simulink model "Slider_Crank_04_auto"  (R2026b)
settings: Solver=ode15s  StopTime=2  MaxStep=0.001  RelTol=1e-5
model workspace (MAT data in the model file):
  Crank_Radius = 0.015
  Crank_Speed = 12.5663706144
  Dead_Volume = 1e-05
  Initial_Tank_Volume = 0.001
  Piston_Area = 0.001
  Piston_Stroke = 0.05
  Pump_Frequency = 2
  Rod_Length = 0.075
  Tank_Area = 0.02
  Valve_Crack_Pressure = 1000
  Valve_Full_Pressure = 10000
undefined symbols (not defined in the file): X, Y, Z
libraries: sm_lib x15, fl_lib x6, nesl_utility x4, SimscapeFluids_lib x3, simulink x1
settings Model: Creator=smiller  LastModifiedBy=smiller
settings SimscapeCC: SimscapeLogType=all  SimscapeNominalValues="[{\"value\":\"1\",\"unit\":\"A\"},{\"value\":\"1\",\"unit\":\"bar\"},{\"value\":\"1\",\"unit\":\"cm^2\"},{\"value\":\"1\",\"unit\":\"cm^3/s\"},{\"value\":\"1\",\"unit\":\"kJ/kg\"},{\"value\":\"1\",\"unit\":\"kW\"},{\"value\":\"1\",\"unit\":\"l\"},{\"value\":\"1\",\"unit\":\"N\"},{\"value\":\"1\",\"unit\":\"N*m\"},{\"value\":\"1\",\"unit\":\"V\"},{\"value\":\"0.001\",\"unit\":\"Wb\"}]"  SimscapeUseEnergyAccounting=off

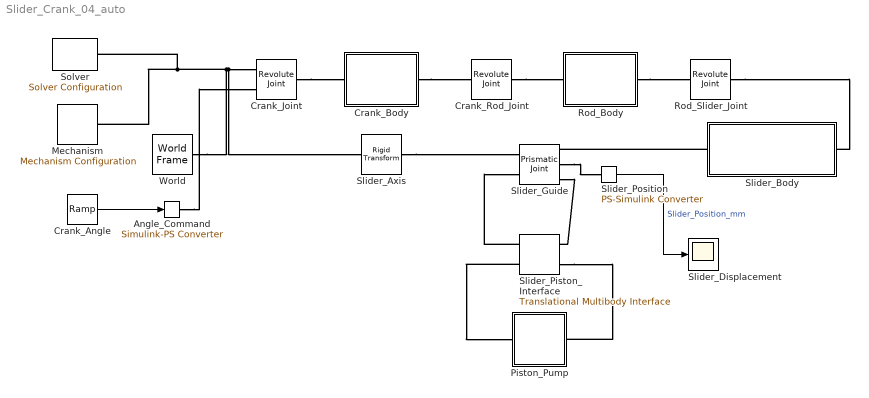
== system Slider_Crank_04_auto ==
  Angle_Command : nesl_utility/Simulink-PS Converter  PhysicalDomain=network_engine_domain  SubClassName=ps_input  LeftPortType=input  RightPortType=output  PseudoPeriodic=off  Frequencies=[]  NoiseDistribution=none  NoiseParameters=[]  Unit=rad  AffineConversion=off  FilteringAndDerivatives=filter  SimscapeFilterOrder=2  InputFilterTimeConstant=0.001  UdotUserProvided=0
  Crank_Angle : simulink/Sources/Ramp  slope=Crank_Speed  start=0  InitialOutput=0
  Crank_Body : Subsystem
  Crank_Joint : sm_lib/Joints/Revolute Joint  JointMode=Normal  CompositeWrenchDir=FollowerOnBase  CompositeWrenchFrame=BaseFrame  SenseConstraintForce=off  SenseConstraintTorque=off  SenseTotalForce=off  SenseTotalTorque=off  PositionTargetSpecify=off  PositionTargetPriority=High  PositionTargetValue=0  PositionTargetValueUnits=deg  VelocityTargetSpecify=off  VelocityTargetPriority=High  VelocityTargetValue=0  VelocityTargetValueUnits=deg/s  EquilibriumPosition=0  EquilibriumPositionUnits=deg  SpringStiffness=0  SpringStiffnessUnits=N*m/deg  DampingCoefficient=0  DampingCoefficientUnits=N*m/(deg/s)  LowerLimitSpecify=off  LowerLimitBound=-90  LowerLimitBoundUnits=deg  LowerLimitStiffness=1e4  LowerLimitStiffnessUnits=N*m/deg  LowerLimitDamping=10  LowerLimitDampingUnits=N*m/(deg/s)  LowerLimitTransitionRegionWidth=0.1  LowerLimitTransitionRegionWidthUnits=deg  UpperLimitSpecify=off  UpperLimitBound=90  UpperLimitBoundUnits=deg  UpperLimitStiffness=1e4  UpperLimitStiffnessUnits=N*m/deg  UpperLimitDamping=10  UpperLimitDampingUnits=N*m/(deg/s)  UpperLimitTransitionRegionWidth=0.1  UpperLimitTransitionRegionWidthUnits=deg  TorqueActuationMode=ComputedTorque  MotionActuationMode=InputMotion  SensePosition=off  SenseVelocity=off  SenseAcceleration=off  SenseTorqueForce=off  SenseLowerLimitTorqueForce=off  SenseUpperLimitTorqueForce=off
  Crank_Rod_Joint : sm_lib/Joints/Revolute Joint  JointMode=Normal  CompositeWrenchDir=FollowerOnBase  CompositeWrenchFrame=BaseFrame  SenseConstraintForce=off  SenseConstraintTorque=off  SenseTotalForce=off  SenseTotalTorque=off  PositionTargetSpecify=off  PositionTargetPriority=High  PositionTargetValue=0  PositionTargetValueUnits=deg  VelocityTargetSpecify=off  VelocityTargetPriority=High  VelocityTargetValue=0  VelocityTargetValueUnits=deg/s  EquilibriumPosition=0  EquilibriumPositionUnits=deg  SpringStiffness=0  SpringStiffnessUnits=N*m/deg  DampingCoefficient=0  DampingCoefficientUnits=N*m/(deg/s)  LowerLimitSpecify=off  LowerLimitBound=-90  LowerLimitBoundUnits=deg  LowerLimitStiffness=1e4  LowerLimitStiffnessUnits=N*m/deg  LowerLimitDamping=10  LowerLimitDampingUnits=N*m/(deg/s)  LowerLimitTransitionRegionWidth=0.1  LowerLimitTransitionRegionWidthUnits=deg  UpperLimitSpecify=off  UpperLimitBound=90  UpperLimitBoundUnits=deg  UpperLimitStiffness=1e4  UpperLimitStiffnessUnits=N*m/deg  UpperLimitDamping=10  UpperLimitDampingUnits=N*m/(deg/s)  UpperLimitTransitionRegionWidth=0.1  UpperLimitTransitionRegionWidthUnits=deg  TorqueActuationMode=NoTorque  MotionActuationMode=ComputedMotion  SensePosition=off  SenseVelocity=off  SenseAcceleration=off  SenseTorqueForce=off  SenseLowerLimitTorqueForce=off  SenseUpperLimitTorqueForce=off
  Mechanism : sm_lib/Utilities/Mechanism Configuration  UniformGravity=Constant  GravityVector=[0 -9.81 0]  GravityVectorUnits=m/s^2  LinearizationDelta=0.001  JointModeTransitionNonlinearIterations=2
  Piston_Pump : Subsystem
  Rod_Body : Subsystem
  Rod_Slider_Joint : sm_lib/Joints/Revolute Joint  JointMode=Normal  CompositeWrenchDir=FollowerOnBase  CompositeWrenchFrame=BaseFrame  SenseConstraintForce=off  SenseConstraintTorque=off  SenseTotalForce=off  SenseTotalTorque=off  PositionTargetSpecify=off  PositionTargetPriority=High  PositionTargetValue=0  PositionTargetValueUnits=deg  VelocityTargetSpecify=off  VelocityTargetPriority=High  VelocityTargetValue=0  VelocityTargetValueUnits=deg/s  EquilibriumPosition=0  EquilibriumPositionUnits=deg  SpringStiffness=0  SpringStiffnessUnits=N*m/deg  DampingCoefficient=0  DampingCoefficientUnits=N*m/(deg/s)  LowerLimitSpecify=off  LowerLimitBound=-90  LowerLimitBoundUnits=deg  LowerLimitStiffness=1e4  LowerLimitStiffnessUnits=N*m/deg  LowerLimitDamping=10  LowerLimitDampingUnits=N*m/(deg/s)  LowerLimitTransitionRegionWidth=0.1  LowerLimitTransitionRegionWidthUnits=deg  UpperLimitSpecify=off  UpperLimitBound=90  UpperLimitBoundUnits=deg  UpperLimitStiffness=1e4  UpperLimitStiffnessUnits=N*m/deg  UpperLimitDamping=10  UpperLimitDampingUnits=N*m/(deg/s)  UpperLimitTransitionRegionWidth=0.1  UpperLimitTransitionRegionWidthUnits=deg  TorqueActuationMode=NoTorque  MotionActuationMode=ComputedMotion  SensePosition=off  SenseVelocity=off  SenseAcceleration=off  SenseTorqueForce=off  SenseLowerLimitTorqueForce=off  SenseUpperLimitTorqueForce=off
  Slider_Axis : sm_lib/Frames and Transforms/Rigid Transform  RotationMethod=StandardAxis  FollAlignAxisA=+X  BaseAlignAxisA=+Y  FollAlignAxisB=+Y  BaseAlignAxisB=+Z  RotationStandardAxis=+Y  RotationAngle=90  RotationAngleUnits=deg  RotationArbitraryAxis=[0 0 1]  RotationSequenceAxes=FollowerAxes  RotationSequence=XYX  RotationSequenceAngles=[0 0 0]  RotationSequenceAnglesUnits=deg  RotationMatrix=[1 0 0;0 1 0;0 0 1]  Quaternion=[1 0 0 0]  TranslationMethod=None  TranslationCartesianOffset=[0 0 0]  TranslationCartesianOffsetUnits=m  TranslationStandardAxis=+Z  TranslationStandardOffset=0  TranslationStandardOffsetUnits=m  TranslationROffset=0  TranslationROffsetUnits=m  TranslationThetaOffset=0  TranslationThetaOffsetUnits=deg  TranslationZOffset=0  TranslationZOffsetUnits=m
  Slider_Body : Subsystem
  Slider_Displacement : Scope
      settings: ActiveDisplayYMinimum=56.250000136812304  ActiveDisplayYMaximum=93.749999984798635
  Slider_Guide : sm_lib/Joints/Prismatic Joint  JointMode=Normal  CompositeWrenchDir=FollowerOnBase  CompositeWrenchFrame=BaseFrame  SenseConstraintForce=off  SenseConstraintTorque=off  SenseTotalForce=off  SenseTotalTorque=off  PositionTargetSpecify=on  PositionTargetPriority=High  PositionTargetValue=Crank_Radius+Rod_Length  PositionTargetValueUnits=m  VelocityTargetSpecify=off  VelocityTargetPriority=High  VelocityTargetValue=0  VelocityTargetValueUnits=m/s  EquilibriumPosition=0  EquilibriumPositionUnits=m  SpringStiffness=0  SpringStiffnessUnits=N/m  DampingCoefficient=0  DampingCoefficientUnits=N/(m/s)  LowerLimitSpecify=off  LowerLimitBound=-1  LowerLimitBoundUnits=m  LowerLimitStiffness=1e6  LowerLimitStiffnessUnits=N/m  LowerLimitDamping=1e3  LowerLimitDampingUnits=N/(m/s)  LowerLimitTransitionRegionWidth=1e-4  LowerLimitTransitionRegionWidthUnits=m  UpperLimitSpecify=off  UpperLimitBound=1  UpperLimitBoundUnits=m  UpperLimitStiffness=1e6  UpperLimitStiffnessUnits=N/m  UpperLimitDamping=1e3  UpperLimitDampingUnits=N/(m/s)  UpperLimitTransitionRegionWidth=1e-4  UpperLimitTransitionRegionWidthUnits=m  TorqueActuationMode=InputTorque  MotionActuationMode=ComputedMotion  SensePosition=on  SenseVelocity=on  SenseAcceleration=off  SenseTorqueForce=off  SenseLowerLimitTorqueForce=off  SenseUpperLimitTorqueForce=off
  Slider_Piston_Interface : fl_lib/Mechanical/Multibody Interfaces/Translational Multibody Interface
  Slider_Position : nesl_utility/PS-Simulink Converter  PhysicalDomain=network_engine_domain  SubClassName=ps_output  LeftPortType=input  RightPortType=output  PseudoPeriodic=off  Frequencies=[]  VectorFormat=inherit  Unit=mm  AffineConversion=off
  Solver : nesl_utility/Solver Configuration  PhysicalDomain=network_engine_domain  SubClassName=solver  LeftPortType=input  RightPortType=generic  Tones=[]  Harmonics=[]  SimulateNoise=off  Profile=off  UseLocalSampling=off  EnableSwitchedLinearOptims=on  FrequencyDomain=off  UseCCode=off  RelTol=0.001  AbsTol=0.001  MinStep=1e-09  ToWorkspace=off  RevertToSquareIcSolve=off  NumHomotopyIterations=100  PhasorMode=off  PhasorModeNumHarmonics=1  ConsistencySolver=NEWTON_XTOL_AFTER_FTOL  CanonicalOrdering=CANONICAL  OptimizeIntermediates=OPTIMIZED  MulticoreSolverChoice=BACKWARD_EULER  IndexReductionMethod=DerivativeReplacement  DoDC=off  ResidualTolerance=1e-09  ConsistencyTolSource=GLOBAL  ConsistencyAbsTol=0.001  ConsistencyRelTol=0.001  ConsistencyTolFactor=0.001  UseLocalSolver=off  LocalSolverChoice=NE_BACKWARD_EULER_ADVANCER  ResolveIndetEquations=on  FunctionEvalNumThread=1  LocalSolverSampleTime=0.001  DoFixedCost=off  MaxNonlinIter=3  MaxModeIter=2  ComputeImpulses=off  ImpulseIterations=2  LinearAlgebra=auto  LinearAlgebraNumThread=0  EquationFormulation=NE_TIME_EF  DelaysMemoryBudget=1024  AutomaticFiltering=on  FilteringTimeConstant=0.001  PartitionStorageMethod=AS_NEEDED  PartitionMemoryBudget=1024  PartitionMethod=BALANCED  MultibodyUseLocalSolver=off  MultibodyLocalSolverChoice=ODE1  MultibodyLocalSolverSampleTime=0.001
  World : sm_lib/Frames and Transforms/World Frame
  wires:
  Crank_Angle/1 -> Angle_Command/1
  Slider_Position/1 -> Slider_Displacement/1  "Slider_Position_mm"
  connections:
  Rod_Body/RConn1 -- Rod_Slider_Joint/LConn1
  World/RConn1 -- Mechanism/RConn1 -- Solver/RConn1 -- Crank_Joint/LConn1 -- Slider_Axis/LConn1
  Slider_Axis/RConn1 -- Slider_Guide/LConn1
  Angle_Command/RConn1 -- Crank_Joint/LConn2
  Crank_Body/RConn1 -- Crank_Rod_Joint/LConn1
  Crank_Joint/RConn1 -- Crank_Body/LConn1
  Crank_Rod_Joint/RConn1 -- Rod_Body/LConn1
  Rod_Slider_Joint/RConn1 -- Slider_Body/LConn1
  Slider_Body/RConn1 -- Slider_Guide/RConn1
  Slider_Guide/RConn2 -- Slider_Position/LConn1
  Slider_Piston_Interface/RConn2 -- Piston_Pump/RConn1
  Slider_Piston_Interface/LConn2 -- Piston_Pump/LConn1
  Slider_Guide/RConn3 -- Slider_Piston_Interface/RConn1
  Slider_Piston_Interface/LConn1 -- Slider_Guide/LConn2

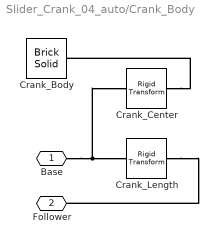
== system Slider_Crank_04_auto/Crank_Body ==
  Crank_Body : sm_lib/Body Elements/Brick Solid  BrickDimensions=[Crank_Radius 0.006 0.006]  BrickDimensionsUnits=m  ExportEntireGeometry=off  InertiaType=CalculateFromGeometry  BasedOnType=Density  Density=1000  DensityUnits=kg/m^3  Mass=1  MassUnits=kg  CenterOfMass=[0 0 0]  CenterOfMassUnits=m  MomentsOfInertia=[1 1 1]  MomentsOfInertiaUnits=kg*m^2  ProductsOfInertia=[0 0 0]  ProductsOfInertiaUnits=kg*m^2  GraphicType=FromGeometry  MarkerShape=Sphere  MarkerSize=10  GraphicVisPropType=SimpleVisualProperties  GraphicDiffuseColor=[0.2 0.5 0.9]  GraphicOpacity=1  GraphicSpecularColor=[0.5 0.5 0.5 1.0]  GraphicAmbientColor=[0.15 0.15 0.15 1.0]  GraphicEmissiveColor=[0.0 0.0 0.0 1.0]  GraphicShininess=75  DoExposeReferenceFrame=on  SerializedFrames=<Frames/>
  Crank_Center : sm_lib/Frames and Transforms/Rigid Transform  RotationMethod=None  FollAlignAxisA=+X  BaseAlignAxisA=+Y  FollAlignAxisB=+Y  BaseAlignAxisB=+Z  RotationStandardAxis=+Z  RotationAngle=0  RotationAngleUnits=deg  RotationArbitraryAxis=[0 0 1]  RotationSequenceAxes=FollowerAxes  RotationSequence=XYX  RotationSequenceAngles=[0 0 0]  RotationSequenceAnglesUnits=deg  RotationMatrix=[1 0 0;0 1 0;0 0 1]  Quaternion=[1 0 0 0]  TranslationMethod=Cartesian  TranslationCartesianOffset=[Crank_Radius/2 0 0]  TranslationCartesianOffsetUnits=m  TranslationStandardAxis=+Z  TranslationStandardOffset=0  TranslationStandardOffsetUnits=m  TranslationROffset=0  TranslationROffsetUnits=m  TranslationThetaOffset=0  TranslationThetaOffsetUnits=deg  TranslationZOffset=0  TranslationZOffsetUnits=m
  Crank_Length : sm_lib/Frames and Transforms/Rigid Transform  RotationMethod=None  FollAlignAxisA=+X  BaseAlignAxisA=+Y  FollAlignAxisB=+Y  BaseAlignAxisB=+Z  RotationStandardAxis=+Z  RotationAngle=0  RotationAngleUnits=deg  RotationArbitraryAxis=[0 0 1]  RotationSequenceAxes=FollowerAxes  RotationSequence=XYX  RotationSequenceAngles=[0 0 0]  RotationSequenceAnglesUnits=deg  RotationMatrix=[1 0 0;0 1 0;0 0 1]  Quaternion=[1 0 0 0]  TranslationMethod=Cartesian  TranslationCartesianOffset=[Crank_Radius 0 0]  TranslationCartesianOffsetUnits=m  TranslationStandardAxis=+Z  TranslationStandardOffset=0  TranslationStandardOffsetUnits=m  TranslationROffset=0  TranslationROffsetUnits=m  TranslationThetaOffset=0  TranslationThetaOffsetUnits=deg  TranslationZOffset=0  TranslationZOffsetUnits=m
  Base : PMIOPort  Side=Left
  Follower : PMIOPort  Port=2  Side=Right
  connections:
  Base/RConn1 -- Crank_Length/LConn1 -- Crank_Center/LConn1
  Crank_Length/RConn1 -- Follower/RConn1
  Crank_Center/RConn1 -- Crank_Body/RConn1

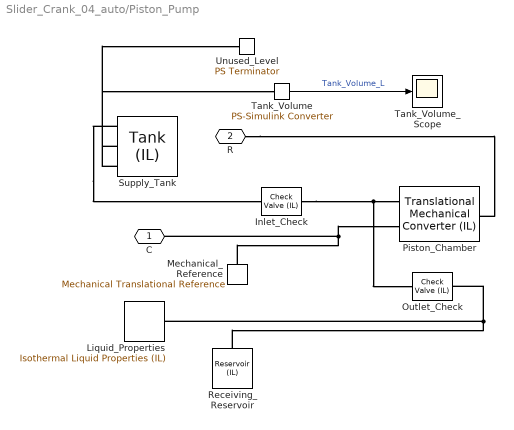
== system Slider_Crank_04_auto/Piston_Pump ==
  Inlet_Check : SimscapeFluids_lib/Isothermal Liquid/Valves & Orifices/Directional Control Valves/Check Valve (IL)  opening_spec=fluids.isothermal_liquid.valves_orifices.enum.PressureOpeningSpec.Linear  pressure_control_spec=fluids.isothermal_liquid.valves_orifices.enum.pressure_control_spec.dp  p_crack_differential=Valve_Crack_Pressure Pa  p_crack_gauge=0.1 MPa  press_max_differential=Valve_Full_Pressure Pa  press_max_gauge=0.2 MPa  area_max=1e-4 m^2  area_leak=1e-10 m^2  p_diff_TLU=[0.01 : 0.01 : 0.1] MPa  valve_area_TLU=[1e-10, 1e-05, 2e-05, 3e-05, 4e-05, 5e-05, 6e-05, 7.5e-05, 8.5e-05, .0001] m^2  vol_flow_TLU=[.000358, .045, .11, .191, .284, .39, .505, .63, .764, .905] .* 1e-3 m^3/s  area=inf m^2  Cd=0.64  Re_c=150  smoothing_factor=0.01  pressure_recovery=false  opening_dynamics=false  tau=0.1 s
  Liquid_Properties : fl_lib/Isothermal Liquid/Utilities/Isothermal Liquid Properties (IL)  rho_L_atm=998.21 kg/m^3  bulk_modulus_model=foundation.enum.bulk_modulus_model.const  beta_gain=6  beta_L_atm=2.1791e9 Pa  nu_atm=1.0034e-6 m^2/s  p_atm=0.101325 MPa  p_min=1 Pa  properties_range_check=simscape.enum.assert.action.error  air_fraction=0.005  polytropic_index=1.0  rho_g_atm=1.225 kg/m^3  air_dissolution_model=false  p_crit=3 MPa
  Mechanical_Reference : fl_lib/Mechanical/Translational Elements/Mechanical Translational Reference
  Outlet_Check : SimscapeFluids_lib/Isothermal Liquid/Valves & Orifices/Directional Control Valves/Check Valve (IL)  opening_spec=fluids.isothermal_liquid.valves_orifices.enum.PressureOpeningSpec.Linear  pressure_control_spec=fluids.isothermal_liquid.valves_orifices.enum.pressure_control_spec.dp  p_crack_differential=Valve_Crack_Pressure Pa  p_crack_gauge=0.1 MPa  press_max_differential=Valve_Full_Pressure Pa  press_max_gauge=0.2 MPa  area_max=1e-4 m^2  area_leak=1e-10 m^2  p_diff_TLU=[0.01 : 0.01 : 0.1] MPa  valve_area_TLU=[1e-10, 1e-05, 2e-05, 3e-05, 4e-05, 5e-05, 6e-05, 7.5e-05, 8.5e-05, .0001] m^2  vol_flow_TLU=[.000358, .045, .11, .191, .284, .39, .505, .63, .764, .905] .* 1e-3 m^3/s  area=inf m^2  Cd=0.64  Re_c=150  smoothing_factor=0.01  pressure_recovery=false  opening_dynamics=false  tau=0.1 s
  Piston_Chamber : fl_lib/Isothermal Liquid/Elements/Translational Mechanical Converter (IL)  mech_orientation=foundation.enum.MechOrientationTranslational.Positive  displacement_spec=foundation.enum.DisplacementSpec.Calculate  x0=2*Crank_Radius m  interface_area=Piston_Area m^2  dead_volume=Dead_Volume m^3  pressure_spec=foundation.enum.pressure_spec.atmospheric  environment_pressure=0.101325 MPa  dynamic_compressibility=true  p0=0.101325 MPa  p_nominal=0.101325 MPa
  Receiving_Reservoir : fl_lib/Isothermal Liquid/Elements/Reservoir (IL)  pressure_input=false  pressure_spec=foundation.enum.pressure_spec.atmospheric  reservoir_pressure=0.101325 MPa
  Supply_Tank : SimscapeFluids_lib/Isothermal Liquid/Tanks & Accumulators/Tank (IL)  num_inlet=fluids.isothermal_liquid.tanks_accumulators.enum.NumInlet.One  pressure_spec=fluids.isothermal_liquid.tanks_accumulators.enum.TankPressureSpec.Atmospheric  tank_pressure=0.101325 MPa  volume_spec=fluids.isothermal_liquid.tanks_accumulators.enum.TankVolumeSpec.Constant  tank_area=Tank_Area m^2  level_TLU=[0, 3, 5] m  volume_TLU=[0, 4, 6] m^3  inlet_height_A=0 m  inlet_area_A=0.01 m^2  inlet_height_AB=[.1, .1] m  inlet_area_AB=[.01, .01] m^2  inlet_height_ABC=[.1, .1, .1] m  inlet_area_ABC=[.01, .01, .01] m^2  inlet_height_ABCD=0.1 * ones(1, 4) m  inlet_area_ABCD=0.01 * ones(1, 4) m^2  inlet_height_ABCDE=0.1 * ones(1, 5) m  inlet_area_ABCDE=0.01 * ones(1, 5) m^2  inlet_height_ABCDEF=0.1 * ones(1, 6) m  inlet_area_ABCDEF=0.01 * ones(1, 6) m^2  level_check=simscape.enum.assert.action.error  capacity_check=simscape.enum.assert.action.none  max_capacity=10 m^3  g=9.81 m/s^2  level_specify=on  level_priority=High  level=Initial_Tank_Volume/Tank_Area m  level_nominal_specify=off  level_nominal_value=1  level_nominal_unit=m  volume_specify=off  volume_priority=High  volume=Initial_Tank_Volume m^3  volume_nominal_specify=off  volume_nominal_value=1  volume_nominal_unit=m^3  mass_specify=off  mass_priority=None  mass=5000 kg  mass_nominal_specify=off  mass_nominal_value=1  mass_nominal_unit=kg
  Tank_Volume : nesl_utility/PS-Simulink Converter  PhysicalDomain=network_engine_domain  SubClassName=ps_output  LeftPortType=input  RightPortType=output  PseudoPeriodic=off  Frequencies=[]  VectorFormat=inherit  Unit=l  AffineConversion=off
  Tank_Volume_Scope : Scope
      settings: ActiveDisplayYMinimum=0.86501519308232389  ActiveDisplayYMaximum=1.01499832083381
  Unused_Level : fl_lib/Physical Signals/Sinks/PS Terminator
  C : PMIOPort  Side=Left
  R : PMIOPort  Port=2  Side=Right
  wires:
  Tank_Volume/1 -> Tank_Volume_Scope/1  "Tank_Volume_L"
  connections:
  Supply_Tank/LConn1 -- Inlet_Check/LConn1
  Supply_Tank/LConn2 -- Tank_Volume/LConn1
  Supply_Tank/LConn3 -- Unused_Level/LConn1
  Receiving_Reservoir/LConn1 -- Outlet_Check/RConn1 -- Liquid_Properties/RConn1
  Inlet_Check/RConn1 -- Piston_Chamber/LConn1 -- Outlet_Check/LConn1
  R/RConn1 -- Piston_Chamber/RConn1
  Mechanical_Reference/LConn1 -- Piston_Chamber/LConn2 -- C/RConn1

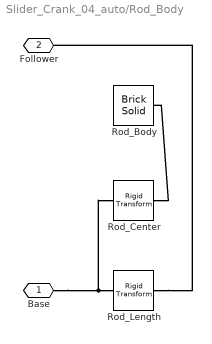
== system Slider_Crank_04_auto/Rod_Body ==
  Rod_Body : sm_lib/Body Elements/Brick Solid  BrickDimensions=[Rod_Length 0.004 0.004]  BrickDimensionsUnits=m  ExportEntireGeometry=off  InertiaType=CalculateFromGeometry  BasedOnType=Density  Density=1000  DensityUnits=kg/m^3  Mass=1  MassUnits=kg  CenterOfMass=[0 0 0]  CenterOfMassUnits=m  MomentsOfInertia=[1 1 1]  MomentsOfInertiaUnits=kg*m^2  ProductsOfInertia=[0 0 0]  ProductsOfInertiaUnits=kg*m^2  GraphicType=FromGeometry  MarkerShape=Sphere  MarkerSize=10  GraphicVisPropType=SimpleVisualProperties  GraphicDiffuseColor=[0.9 0.6 0.15]  GraphicOpacity=1  GraphicSpecularColor=[0.5 0.5 0.5 1.0]  GraphicAmbientColor=[0.15 0.15 0.15 1.0]  GraphicEmissiveColor=[0.0 0.0 0.0 1.0]  GraphicShininess=75  DoExposeReferenceFrame=on  SerializedFrames=<Frames/>
  Rod_Center : sm_lib/Frames and Transforms/Rigid Transform  RotationMethod=None  FollAlignAxisA=+X  BaseAlignAxisA=+Y  FollAlignAxisB=+Y  BaseAlignAxisB=+Z  RotationStandardAxis=+Z  RotationAngle=0  RotationAngleUnits=deg  RotationArbitraryAxis=[0 0 1]  RotationSequenceAxes=FollowerAxes  RotationSequence=XYX  RotationSequenceAngles=[0 0 0]  RotationSequenceAnglesUnits=deg  RotationMatrix=[1 0 0;0 1 0;0 0 1]  Quaternion=[1 0 0 0]  TranslationMethod=Cartesian  TranslationCartesianOffset=[Rod_Length/2 0 0]  TranslationCartesianOffsetUnits=m  TranslationStandardAxis=+Z  TranslationStandardOffset=0  TranslationStandardOffsetUnits=m  TranslationROffset=0  TranslationROffsetUnits=m  TranslationThetaOffset=0  TranslationThetaOffsetUnits=deg  TranslationZOffset=0  TranslationZOffsetUnits=m
  Rod_Length : sm_lib/Frames and Transforms/Rigid Transform  RotationMethod=None  FollAlignAxisA=+X  BaseAlignAxisA=+Y  FollAlignAxisB=+Y  BaseAlignAxisB=+Z  RotationStandardAxis=+Z  RotationAngle=0  RotationAngleUnits=deg  RotationArbitraryAxis=[0 0 1]  RotationSequenceAxes=FollowerAxes  RotationSequence=XYX  RotationSequenceAngles=[0 0 0]  RotationSequenceAnglesUnits=deg  RotationMatrix=[1 0 0;0 1 0;0 0 1]  Quaternion=[1 0 0 0]  TranslationMethod=Cartesian  TranslationCartesianOffset=[Rod_Length 0 0]  TranslationCartesianOffsetUnits=m  TranslationStandardAxis=+Z  TranslationStandardOffset=0  TranslationStandardOffsetUnits=m  TranslationROffset=0  TranslationROffsetUnits=m  TranslationThetaOffset=0  TranslationThetaOffsetUnits=deg  TranslationZOffset=0  TranslationZOffsetUnits=m
  Base : PMIOPort  Side=Left
  Follower : PMIOPort  Port=2  Side=Right
  connections:
  Rod_Length/RConn1 -- Follower/RConn1
  Rod_Center/RConn1 -- Rod_Body/RConn1
  Rod_Length/LConn1 -- Base/RConn1 -- Rod_Center/LConn1

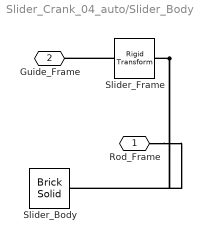
== system Slider_Crank_04_auto/Slider_Body ==
  Slider_Body : sm_lib/Body Elements/Brick Solid  BrickDimensions=[0.012 0.012 0.012]  BrickDimensionsUnits=m  ExportEntireGeometry=off  InertiaType=CalculateFromGeometry  BasedOnType=Density  Density=1000  DensityUnits=kg/m^3  Mass=1  MassUnits=kg  CenterOfMass=[0 0 0]  CenterOfMassUnits=m  MomentsOfInertia=[1 1 1]  MomentsOfInertiaUnits=kg*m^2  ProductsOfInertia=[0 0 0]  ProductsOfInertiaUnits=kg*m^2  GraphicType=FromGeometry  MarkerShape=Sphere  MarkerSize=10  GraphicVisPropType=SimpleVisualProperties  GraphicDiffuseColor=[0.3 0.7 0.4]  GraphicOpacity=1  GraphicSpecularColor=[0.5 0.5 0.5 1.0]  GraphicAmbientColor=[0.15 0.15 0.15 1.0]  GraphicEmissiveColor=[0.0 0.0 0.0 1.0]  GraphicShininess=75  DoExposeReferenceFrame=on  SerializedFrames=<Frames/>
  Slider_Frame : sm_lib/Frames and Transforms/Rigid Transform  RotationMethod=StandardAxis  FollAlignAxisA=+X  BaseAlignAxisA=+Y  FollAlignAxisB=+Y  BaseAlignAxisB=+Z  RotationStandardAxis=+Y  RotationAngle=-90  RotationAngleUnits=deg  RotationArbitraryAxis=[0 0 1]  RotationSequenceAxes=FollowerAxes  RotationSequence=XYX  RotationSequenceAngles=[0 0 0]  RotationSequenceAnglesUnits=deg  RotationMatrix=[1 0 0;0 1 0;0 0 1]  Quaternion=[1 0 0 0]  TranslationMethod=None  TranslationCartesianOffset=[0 0 0]  TranslationCartesianOffsetUnits=m  TranslationStandardAxis=+Z  TranslationStandardOffset=0  TranslationStandardOffsetUnits=m  TranslationROffset=0  TranslationROffsetUnits=m  TranslationThetaOffset=0  TranslationThetaOffsetUnits=deg  TranslationZOffset=0  TranslationZOffsetUnits=m
  Rod_Frame : PMIOPort  Side=Left
  Guide_Frame : PMIOPort  Port=2  Side=Right
  connections:
  Slider_Frame/LConn1 -- Guide_Frame/RConn1
  Slider_Frame/RConn1 -- Slider_Body/RConn1 -- Rod_Frame/RConn1
